simulink model "L2_scheme"  (R2026b)
settings: Solver=VariableStepAuto
settings Model: Creator=Anna  LastModifiedBy=Anna
settings DebuggingCC: AlgebraicLoopMsg=none

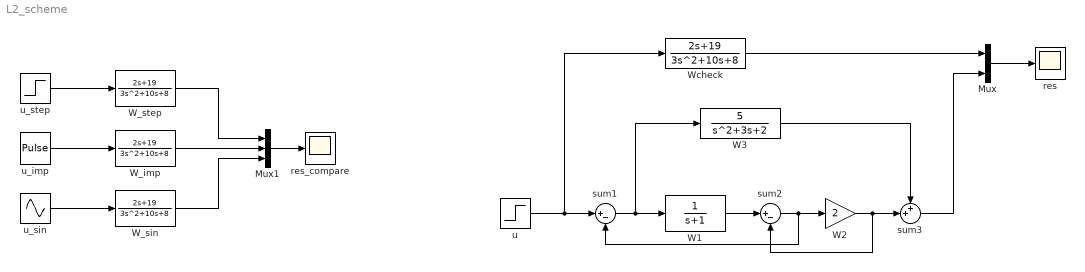
== system L2_scheme ==
  " W_sin" : TransferFcn  Numerator=[2 19]  Denominator=[3 10 8]
  Mux : Mux  Inputs=2
  Mux1 : Mux  Inputs=3
  W1 : TransferFcn  Denominator=[1 1]
  W2 : Gain  Gain=2
  W3 : TransferFcn  Numerator=[5]  Denominator=[1 3 2]
  "W_imp " : TransferFcn  Numerator=[2 19]  Denominator=[3 10 8]
  "W_step " : TransferFcn  Numerator=[2 19]  Denominator=[3 10 8]
  Wcheck : TransferFcn  Numerator=[2 19]  Denominator=[3 10 8]
  res : Scope
      settings: ActiveDisplayYMinimum=-1.0607213546742169  ActiveDisplayYMaximum=3.5447114197657079
  res_compare : Scope
      settings: ActiveDisplayYMinimum=-3.11155336256629  ActiveDisplayYMaximum=3.3925341661637898
  sum1 : Sum  Inputs=|+-
  sum2 : Sum  Inputs=|+-
  sum3 : Sum  Inputs=++|
  u : Step  SampleTime=0
  "u_imp " : DiscretePulseGenerator  PulseType=Time based  Period=10  PulseWidth=5
  "u_sin " : Sin  SampleTime=0
  u_step : Step  SampleTime=0
  wires:
  sum1/1 -> W3/1, W1/1
  W1/1 -> sum2/1
  sum2/1 -> sum1/2, W2/1
  W2/1 -> sum2/2, sum3/2
  W3/1 -> sum3/1
  Mux/1 -> res/1
  sum3/1 -> Mux/2
  Wcheck/1 -> Mux/1
  u/1 -> Wcheck/1, sum1/1
  "W_step "/1 -> Mux1/1
  u_step/1 -> "W_step "/1
  Mux1/1 -> res_compare/1
  " W_sin"/1 -> Mux1/3
  "u_imp "/1 -> "W_imp "/1
  "u_sin "/1 -> " W_sin"/1
  "W_imp "/1 -> Mux1/2
